simulink model "Buck_Parallel"  (R2023b)
settings: Solver=VariableStepAuto  StartTime=0.0  StopTime=0.03  RelTol=1e-3
libraries: spsSeriesRLCBranchLib x12, spsMosfetLib x11, spsCurrentMeasurementLib x9, simulink x6, spsVoltageMeasurementLib x6, slpidlib x6, spsDCVoltageSourceLib x2, spsControlledCurrentSourceLib x2, spsMeanLib x1, spsRMSLib x1, spspowerguiLib x1
settings Model: SimulationMode=accelerator  Creator=45276  LastModifiedBy=Epiphanye

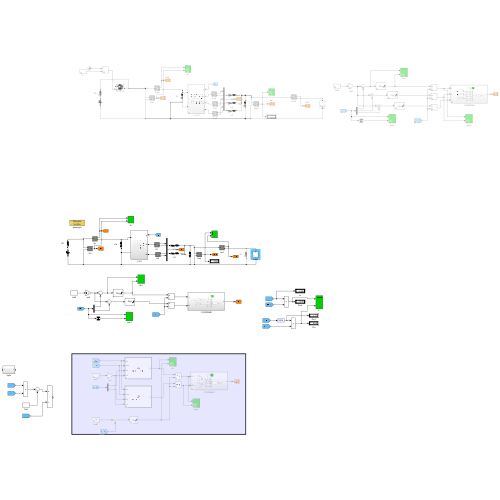
[thumbnail: Simulink's stored preview of the top-level diagram]
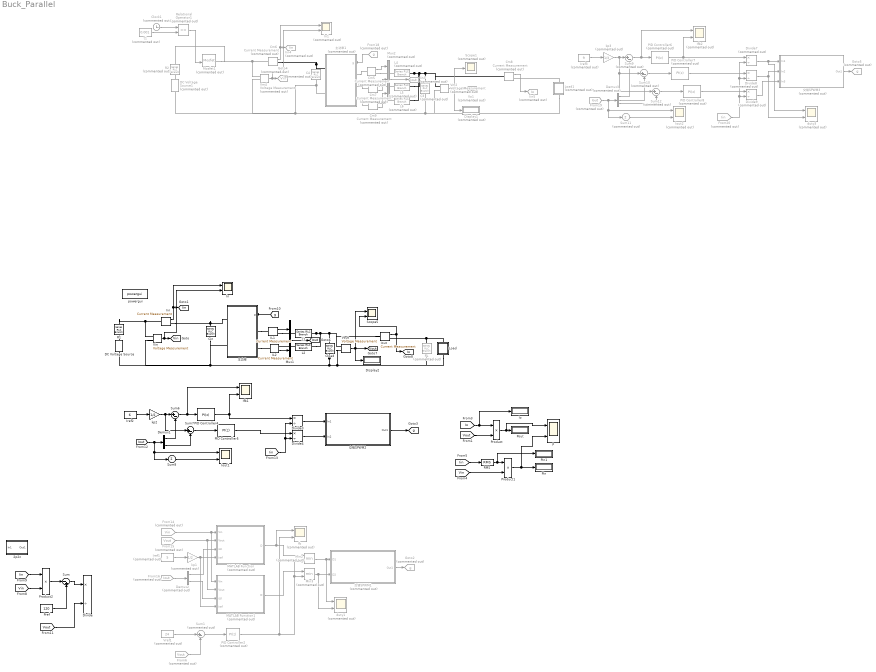
== system Buck_Parallel ==
  2p2z : Subsystem
  C3 : spsSeriesRLCBranchLib/Series RLC Branch  Commented=on  LConnTagsString=__new0  RConnTagsString=__new0  BranchType=RC  Resistance=0.015  Inductance=0  SetiL0=off  InitialCurrent=0  Capacitance=100e-6  Setx0=on  InitialVoltage=18  Measurements=None
  C4 : spsSeriesRLCBranchLib/Series RLC Branch  Commented=on  LConnTagsString=__new0  RConnTagsString=__new0  BranchType=RC  Resistance=0.01  Inductance=0  SetiL0=off  InitialCurrent=0  Capacitance=10e-6  Setx0=on  InitialVoltage=24  Measurements=None
  Cin : spsSeriesRLCBranchLib/Series RLC Branch  LConnTagsString=__new0  RConnTagsString=__new0  BranchType=RC  Resistance=0.15  Inductance=0  SetiL0=off  InitialCurrent=0  Capacitance=81e-6  Setx0=on  InitialVoltage=24  Measurements=None
  Cload : spsSeriesRLCBranchLib/Series RLC Branch  LConnTagsString=__new0  RConnTagsString=__new0  BranchType=RC  Resistance=0.018  Inductance=0  SetiL0=off  InitialCurrent=0  Capacitance=440e-6  Setx0=on  InitialVoltage=0  Measurements=None
  Clock1 : Clock  Commented=on
  Cm{5..9} (5 alike) : spsCurrentMeasurementLib/Current Measurement  Commented=on  PhasorSimulation=off  OutputType=Complex  PSBequivalent=0
  DC Voltage Source : spsDCVoltageSourceLib/DC Voltage Source  Amplitude=24  Measurements=None
  DC Voltage Source1 : spsDCVoltageSourceLib/DC Voltage Source  Commented=on  Amplitude=60  Measurements=None
  Demux1 : Demux  Outputs=2
  Demux2 : Demux  Commented=on  Outputs=2
  Demux3 : Demux  Commented=on  Outputs=3
  Display1 : Display  Commented=on
  Display2 : Display
  Divide : Product  Inputs=*/
  Divide3 : Product  Inputs=*/
  Divide4 : Product  Inputs=*/
  Divide7 : Product  Commented=on  Inputs=*/
  Divide8 : Product  Commented=on  Inputs=*/
  Divide9 : Product  Commented=on  Inputs=*/
  From14 : From  Commented=on  GotoTag=Vin  TagVisibility=global
      settings: CloseFcn=tagdialog Close
  From15 : From  Commented=on  GotoTag=Vout  TagVisibility=global
      settings: CloseFcn=tagdialog Close
  From16 : From  Commented=on  GotoTag=Iout  TagVisibility=global
      settings: CloseFcn=tagdialog Close
  From18 : From  Commented=on  GotoTag=g  TagVisibility=global
      settings: CloseFcn=tagdialog Close
  From19 : From  Commented=on  GotoTag=Iout  TagVisibility=global
      settings: CloseFcn=tagdialog Close
  From20 : From  Commented=on  GotoTag=Iin  TagVisibility=global
      settings: CloseFcn=tagdialog Close
  From6 : From  Commented=on  GotoTag=Vout  TagVisibility=global
      settings: CloseFcn=tagdialog Close
  Goto2 : Goto  Commented=on  GotoTag=g  TagVisibility=global
  Goto4 : Goto  Commented=on  GotoTag=Vin  TagVisibility=global
  Goto5 : Goto  Commented=on  GotoTag=g  TagVisibility=global
  IL1 : spsCurrentMeasurementLib/Current Measurement  PhasorSimulation=off  OutputType=Complex  PSBequivalent=0
  IL2 : spsCurrentMeasurementLib/Current Measurement  PhasorSimulation=off  OutputType=Complex  PSBequivalent=0
  Ifb1 : Scope  NumInputPorts=2
  Ifb2 : Scope  Commented=on  NumInputPorts=2
  Iin : spsCurrentMeasurementLib/Current Measurement  PhasorSimulation=off  OutputType=Complex  PSBequivalent=0
  Iin3 : Goto  Commented=on  GotoTag=Iout  TagVisibility=global
  Iin4 : Goto  Commented=on  GotoTag=Iin  TagVisibility=global
  Iin5 : Goto  Commented=on  GotoTag=Io  TagVisibility=global
  In : Scope  NumInputPorts=2
  In1 : Scope  Commented=on  NumInputPorts=2
  Io : Display
  Iout : spsCurrentMeasurementLib/Current Measurement  PhasorSimulation=off  OutputType=Complex  PSBequivalent=0
  Iout1 : Scope  NumInputPorts=2
  Iout2 : Scope  Commented=on  NumInputPorts=2
  Iref1 : Constant  Commented=on  Value=5
  Iref2 : Constant  Value=6
  Iref3 : Constant  Commented=on  Value=9
  L1 : spsSeriesRLCBranchLib/Series RLC Branch  LConnTagsString=__new0  RConnTagsString=__new0  BranchType=RL  Resistance=0.04  Inductance=221e-6  SetiL0=off  InitialCurrent=0  Capacitance=inf  Setx0=off  InitialVoltage=0  Measurements=None
  L2 : spsSeriesRLCBranchLib/Series RLC Branch  LConnTagsString=__new0  RConnTagsString=__new0  BranchType=RL  Resistance=0.04  Inductance=218e-6  SetiL0=off  InitialCurrent=0  Capacitance=inf  Setx0=off  InitialVoltage=0  Measurements=None
  L4 : spsSeriesRLCBranchLib/Series RLC Branch  Commented=on  LConnTagsString=__new0  RConnTagsString=__new0  BranchType=RL  Resistance=0.1  Inductance=4e-5  SetiL0=off  InitialCurrent=0  Capacitance=inf  Setx0=off  InitialVoltage=0  Measurements=None
  L5 : spsSeriesRLCBranchLib/Series RLC Branch  Commented=on  LConnTagsString=__new0  RConnTagsString=__new0  BranchType=RL  Resistance=0.1  Inductance=4e-5  SetiL0=off  InitialCurrent=0  Capacitance=inf  Setx0=off  InitialVoltage=0  Measurements=None
  L6 : spsSeriesRLCBranchLib/Series RLC Branch  Commented=on  LConnTagsString=__new0  RConnTagsString=__new0  BranchType=RL  Resistance=0.1  Inductance=4e-5  SetiL0=off  InitialCurrent=0  Capacitance=inf  Setx0=off  InitialVoltage=0  Measurements=None
  Load : Subsystem  mask{Vst1=[2 2 1 1 0.5 0.5].', Tst1=[0 0.01 0.01+eps 0.02 0.02+eps 0.03].', Tstsp=1e-8}
      mask prompts: Vst1 "突变值Vst1, eg:[3 3 8 8 2 2].'"; Tst1 "突变时间Tst1, eg:[0 0.01 0.01+eps 0.02 0.02+eps 0.03].'"; Tstsp "采样时间Tstsp"
      settings: PortSchema="{\"entries\":[{\"content\":{\"sides\":[{\"content\":{},\"type\":\"ConnectorPlacement.EquallySpacedRectSide\",\"uuid\":\"4352356a-a73d-4efd-aeba-c61bfc863045\"},{\"content\":{\"side\":\"RIGHT\"},\"type\":\"ConnectorPlacement.EquallySpacedRectSide\",\"uuid\":\"a043c14f-179e-462d-8cc8-5b83a7edcd21\"},{\"content\":{\"connectorIds\":[\"LConn1\"],\"side\":\"TOP\"},\"type\":\"ConnectorPlacement.EquallySpacedRectSide\",\"uuid\":\"f8810edc-586f-49c6-95ea-bd3a7aa2b56d\"},{\"content\":{\"connectorIds\":[\"RConn1\"],\"side\":\"BOTTOM\"},\"type\":\"ConnectorPlacement.EquallySpacedRectSide\",\"uuid\":\"956d2570-7b82-4c39-8513-d9bfab6f6be6\"}]},\"type\":\"ConnectorPlacement.EquallySpacedConnector\",\"uuid\":\"2f028cb1-1f36-487b-8c9b-3c22934b1877\"}],\"packageUris\":[\"http://schema.mathworks.com/mf0/Connector/R2020b\"],\"version\":\"1.0\"}"
      mask DialogControl ParameterGroupVar Prompt: 参数
  Load1 : Subsystem  Commented=on  mask{Vst1=[3 3 8 8 2 2].', Tst1=[0 0.01 0.01+eps 0.02 0.02+eps 0.03].', Tstsp=1e-8}
      mask prompts: Vst1 "突变值Vst1, eg:[3 3 8 8 2 2].'"; Tst1 "突变时间Tst1, eg:[0 0.01 0.01+eps 0.02 0.02+eps 0.03].'"; Tstsp "采样时间Tstsp"
      settings: PortSchema="{\"entries\":[{\"content\":{\"sides\":[{\"content\":{},\"type\":\"ConnectorPlacement.EquallySpacedRectSide\",\"uuid\":\"4352356a-a73d-4efd-aeba-c61bfc863045\"},{\"content\":{\"side\":\"RIGHT\"},\"type\":\"ConnectorPlacement.EquallySpacedRectSide\",\"uuid\":\"a043c14f-179e-462d-8cc8-5b83a7edcd21\"},{\"content\":{\"connectorIds\":[\"LConn1\"],\"side\":\"TOP\"},\"type\":\"ConnectorPlacement.EquallySpacedRectSide\",\"uuid\":\"f8810edc-586f-49c6-95ea-bd3a7aa2b56d\"},{\"content\":{\"connectorIds\":[\"RConn1\"],\"side\":\"BOTTOM\"},\"type\":\"ConnectorPlacement.EquallySpacedRectSide\",\"uuid\":\"956d2570-7b82-4c39-8513-d9bfab6f6be6\"}]},\"type\":\"ConnectorPlacement.EquallySpacedConnector\",\"uuid\":\"2f028cb1-1f36-487b-8c9b-3c22934b1877\"}],\"packageUris\":[\"http://schema.mathworks.com/mf0/Connector/R2020b\"],\"version\":\"1.0\"}"
      mask DialogControl ParameterGroupVar Prompt: 参数
  MATLAB Function : MATLAB Function  Commented=on  TreatAsAtomicUnit=on
  MATLAB Function1 : MATLAB Function  Commented=on  TreatAsAtomicUnit=on
  Min2 : MinMax  Commented=on  Inputs=2
  Min3 : MinMax  Commented=on  Inputs=2
  Mosfet1 : spsMosfetLib/Mosfet  Commented=on  Ron=0.1  Lon=0  Rd=0.01  Vfd=0  IC=0  Rs=1e5  Cs=inf  Measurements=off
  Mux1 : Mux  Inputs=2
  Mux2 : Mux  Commented=on  Inputs=3
  P : Scope  NumInputPorts=2
  PID Controller2 : slpidlib/PID Controller  Commented=on  Controller=PI  Form=Parallel  TimeDomain=Discrete-time  UseExternalTs=off  SampleTime=-1  IntegratorMethod=Forward Euler  FilterMethod=Forward Euler  ControllerParametersSource=internal  P=1.45  I=15  UseKiTs=off  D=0  N=100  UseFilter=on  TunerSelectOption=Transfer Function Based (PID Tuner App)  InitialConditionSource=internal  InitialConditionForIntegrator=0  InitialConditionForFilter=0  DifferentiatorICPrevScaledInput=0  ExternalReset=none  TrackingMode=off  Kt=100  LimitOutput=on  SatLimitsSource=internal  UpperSaturationLimit=1  LowerSaturationLimit=0  LinearizeAsGain=on  AntiWindupMode=clamping  Kb=1  LimitIntegrator=off  UpperIntegratorSaturationLimit=0.95  LowerIntegratorSaturationLimit=0  POutMin=[]  POutMax=[]  IOutMin=[]  IOutMax=[]  DOutMin=[]  DOutMax=[]  NOutMin=[]  NOutMax=[]  SumOutMin=[]  SumOutMax=[]  SaturationOutMin=[]  SaturationOutMax=[]  PParamMin=[]  PParamMax=[]  IParamMin=[]  IParamMax=[]  DParamMin=[]  DParamMax=[]  NParamMin=[]  NParamMax=[]  KbParamMin=[]  KbParamMax=[]  KtParamMin=[]  KtParamMax=[]  KbOutMin=[]  KbOutMax=[]  KtOutMin=[]  KtOutMax=[]  IntegratorOutMin=[]  IntegratorOutMax=[]  FilterOutMin=[]  FilterOutMax=[]  SumI1OutMin=[]  SumI1OutMax=[]  SumI2OutMin=[]  SumI2OutMax=[]  SumI3OutMin=[]  SumI3OutMax=[]  SumI4OutMin=[]  SumI4OutMax=[]  SumDOutMin=[]  SumDOutMax=[]  DifferentiatorOutMin=[]  DifferentiatorOutMax=[]  FilterDiffOutCoefMin=[]  FilterDiffOutCoefMax=[]  ReciprocalOutMin=[]  ReciprocalOutMax=[]  SumDenOutMin=[]  SumDenOutMax=[]  SumNumOutMin=[]  SumNumOutMax=[]  DivideOutMin=[]  DivideOutMax=[]  UdiffTsProdOutMin=[]  UdiffTsProdOutMax=[]  NTsProdOutMin=[]  NTsProdOutMax=[]  UintegralTsProdOutMin=[]  UintegralTsProdOutMax=[]  UngainTsProdOutMin=[]  UngainTsProdOutMax=[]  ClampingZeroOutDataTypeStr=Inherit: Inherit via back propagation  ClampingZeroOutMin=[]  ClampingZeroOutMax=[]  FilterDenConstantOutDataTypeStr=Inherit: Inherit via back propagation  FilterDenConstantOutMin=[]  FilterDenConstantOutMax=[]  PCopyOutDataTypeStr=Inherit: Inherit via back propagation  PCopyOutMin=[]  PCopyOutMax=[]  NCopyOutDataTypeStr=Inherit: Inherit via back propagation  NCopyOutMin=[]  NCopyOutMax=[]  IntegratorContinuousStateAttributes=''  IntegratorStateMustResolveToSignalObject=off  IntegratorRTWStateStorageClass=Auto  FilterContinuousStateAttributes=''  FilterStateMustResolveToSignalObject=off  FilterRTWStateStorageClass=Auto  ParallelPVariant=InternalParameters  IdealPVariant=Disabled  IVariant=InternalParameters  DVariant=Disabled  IntegratorVariant=Discrete  SatVariant=Enabled  AWVariant=DiscClampingParallel  PCopyVariant=Disabled  TRVariant=Disabled  FdbkBlocksVariant=Forward  IdealPFdbkVariant=Disabled  SatFdbkVariant=Disabled  DerivativeFilterVariant=Disabled  NVariant=Disabled  NCopyVariant=Disabled_SignalSpec  FilterICVariant=Disabled  IntegratorICVariant=InternalICs  ExternalResetVariant=Disabled  TRSumVariant=Passthrough  SumFdbkVariant=Disabled  SumVariant=Sum_PI  TsampFilterVariant=InternalTs  TsampNgainVariant=Passthrough  TsampIntegralVariant=Disabled_SignalSpec  ExternalSaturationOutDataTypeStr=Inherit: Same as second input
  PID Controller4 : slpidlib/PID Controller  Controller=PI  Form=Parallel  TimeDomain=Discrete-time  UseExternalTs=off  SampleTime=-1  IntegratorMethod=Forward Euler  FilterMethod=Forward Euler  ControllerParametersSource=internal  P=0.032  I=160  UseKiTs=off  D=0  N=100  UseFilter=on  TunerSelectOption=Transfer Function Based (PID Tuner App)  InitialConditionSource=internal  InitialConditionForIntegrator=0  InitialConditionForFilter=0  DifferentiatorICPrevScaledInput=0  ExternalReset=none  TrackingMode=off  Kt=1  LimitOutput=on  SatLimitsSource=internal  UpperSaturationLimit=1  LowerSaturationLimit=0  LinearizeAsGain=off  AntiWindupMode=clamping  Kb=1  LimitIntegrator=off  UpperIntegratorSaturationLimit=inf  LowerIntegratorSaturationLimit=-inf  POutMin=[]  POutMax=[]  IOutMin=[]  IOutMax=[]  DOutMin=[]  DOutMax=[]  NOutMin=[]  NOutMax=[]  SumOutMin=[]  SumOutMax=[]  SaturationOutMin=[]  SaturationOutMax=[]  PParamMin=[]  PParamMax=[]  IParamMin=[]  IParamMax=[]  DParamMin=[]  DParamMax=[]  NParamMin=[]  NParamMax=[]  KbParamMin=[]  KbParamMax=[]  KtParamMin=[]  KtParamMax=[]  KbOutMin=[]  KbOutMax=[]  KtOutMin=[]  KtOutMax=[]  IntegratorOutMin=[]  IntegratorOutMax=[]  FilterOutMin=[]  FilterOutMax=[]  SumI1OutMin=[]  SumI1OutMax=[]  SumI2OutMin=[]  SumI2OutMax=[]  SumI3OutMin=[]  SumI3OutMax=[]  SumI4OutMin=[]  SumI4OutMax=[]  SumDOutMin=[]  SumDOutMax=[]  DifferentiatorOutMin=[]  DifferentiatorOutMax=[]  FilterDiffOutCoefMin=[]  FilterDiffOutCoefMax=[]  ReciprocalOutMin=[]  ReciprocalOutMax=[]  SumDenOutMin=[]  SumDenOutMax=[]  SumNumOutMin=[]  SumNumOutMax=[]  DivideOutMin=[]  DivideOutMax=[]  UdiffTsProdOutMin=[]  UdiffTsProdOutMax=[]  NTsProdOutMin=[]  NTsProdOutMax=[]  UintegralTsProdOutMin=[]  UintegralTsProdOutMax=[]  UngainTsProdOutMin=[]  UngainTsProdOutMax=[]  ClampingZeroOutDataTypeStr=Inherit: Inherit via back propagation  ClampingZeroOutMin=[]  ClampingZeroOutMax=[]  FilterDenConstantOutDataTypeStr=Inherit: Inherit via back propagation  FilterDenConstantOutMin=[]  FilterDenConstantOutMax=[]  PCopyOutDataTypeStr=Inherit: Inherit via back propagation  PCopyOutMin=[]  PCopyOutMax=[]  NCopyOutDataTypeStr=Inherit: Inherit via back propagation  NCopyOutMin=[]  NCopyOutMax=[]  IntegratorContinuousStateAttributes=''  IntegratorStateMustResolveToSignalObject=off  IntegratorRTWStateStorageClass=Auto  FilterContinuousStateAttributes=''  FilterStateMustResolveToSignalObject=off  FilterRTWStateStorageClass=Auto  ParallelPVariant=InternalParameters  IdealPVariant=Disabled  IVariant=InternalParameters  DVariant=Disabled  IntegratorVariant=Discrete  SatVariant=Enabled  AWVariant=DiscClampingParallel  PCopyVariant=Disabled  TRVariant=Disabled  FdbkBlocksVariant=Forward  IdealPFdbkVariant=Disabled  SatFdbkVariant=Disabled  DerivativeFilterVariant=Disabled  NVariant=Disabled  NCopyVariant=Disabled_SignalSpec  FilterICVariant=Disabled  IntegratorICVariant=InternalICs  ExternalResetVariant=Disabled  TRSumVariant=Passthrough  SumFdbkVariant=Disabled  SumVariant=Sum_PI  TsampFilterVariant=InternalTs  TsampNgainVariant=Passthrough  TsampIntegralVariant=Disabled_SignalSpec  ExternalSaturationOutDataTypeStr=Inherit: Same as second input
  PID Controller5 : slpidlib/PID Controller  Controller=PI  Form=Parallel  TimeDomain=Discrete-time  UseExternalTs=off  SampleTime=-1  IntegratorMethod=Forward Euler  FilterMethod=Forward Euler  ControllerParametersSource=internal  P=0.032  I=160  UseKiTs=off  D=0  N=100  UseFilter=on  TunerSelectOption=Transfer Function Based (PID Tuner App)  InitialConditionSource=internal  InitialConditionForIntegrator=0  InitialConditionForFilter=0  DifferentiatorICPrevScaledInput=0  ExternalReset=none  TrackingMode=off  Kt=1  LimitOutput=on  SatLimitsSource=internal  UpperSaturationLimit=1  LowerSaturationLimit=0  LinearizeAsGain=off  AntiWindupMode=clamping  Kb=1  LimitIntegrator=off  UpperIntegratorSaturationLimit=inf  LowerIntegratorSaturationLimit=-inf  POutMin=[]  POutMax=[]  IOutMin=[]  IOutMax=[]  DOutMin=[]  DOutMax=[]  NOutMin=[]  NOutMax=[]  SumOutMin=[]  SumOutMax=[]  SaturationOutMin=[]  SaturationOutMax=[]  PParamMin=[]  PParamMax=[]  IParamMin=[]  IParamMax=[]  DParamMin=[]  DParamMax=[]  NParamMin=[]  NParamMax=[]  KbParamMin=[]  KbParamMax=[]  KtParamMin=[]  KtParamMax=[]  KbOutMin=[]  KbOutMax=[]  KtOutMin=[]  KtOutMax=[]  IntegratorOutMin=[]  IntegratorOutMax=[]  FilterOutMin=[]  FilterOutMax=[]  SumI1OutMin=[]  SumI1OutMax=[]  SumI2OutMin=[]  SumI2OutMax=[]  SumI3OutMin=[]  SumI3OutMax=[]  SumI4OutMin=[]  SumI4OutMax=[]  SumDOutMin=[]  SumDOutMax=[]  DifferentiatorOutMin=[]  DifferentiatorOutMax=[]  FilterDiffOutCoefMin=[]  FilterDiffOutCoefMax=[]  ReciprocalOutMin=[]  ReciprocalOutMax=[]  SumDenOutMin=[]  SumDenOutMax=[]  SumNumOutMin=[]  SumNumOutMax=[]  DivideOutMin=[]  DivideOutMax=[]  UdiffTsProdOutMin=[]  UdiffTsProdOutMax=[]  NTsProdOutMin=[]  NTsProdOutMax=[]  UintegralTsProdOutMin=[]  UintegralTsProdOutMax=[]  UngainTsProdOutMin=[]  UngainTsProdOutMax=[]  ClampingZeroOutDataTypeStr=Inherit: Inherit via back propagation  ClampingZeroOutMin=[]  ClampingZeroOutMax=[]  FilterDenConstantOutDataTypeStr=Inherit: Inherit via back propagation  FilterDenConstantOutMin=[]  FilterDenConstantOutMax=[]  PCopyOutDataTypeStr=Inherit: Inherit via back propagation  PCopyOutMin=[]  PCopyOutMax=[]  NCopyOutDataTypeStr=Inherit: Inherit via back propagation  NCopyOutMin=[]  NCopyOutMax=[]  IntegratorContinuousStateAttributes=''  IntegratorStateMustResolveToSignalObject=off  IntegratorRTWStateStorageClass=Auto  FilterContinuousStateAttributes=''  FilterStateMustResolveToSignalObject=off  FilterRTWStateStorageClass=Auto  ParallelPVariant=InternalParameters  IdealPVariant=Disabled  IVariant=InternalParameters  DVariant=Disabled  IntegratorVariant=Discrete  SatVariant=Enabled  AWVariant=DiscClampingParallel  PCopyVariant=Disabled  TRVariant=Disabled  FdbkBlocksVariant=Forward  IdealPFdbkVariant=Disabled  SatFdbkVariant=Disabled  DerivativeFilterVariant=Disabled  NVariant=Disabled  NCopyVariant=Disabled_SignalSpec  FilterICVariant=Disabled  IntegratorICVariant=InternalICs  ExternalResetVariant=Disabled  TRSumVariant=Passthrough  SumFdbkVariant=Disabled  SumVariant=Sum_PI  TsampFilterVariant=InternalTs  TsampNgainVariant=Passthrough  TsampIntegralVariant=Disabled_SignalSpec  ExternalSaturationOutDataTypeStr=Inherit: Same as second input
  PID Controller6 : slpidlib/PID Controller  Commented=on  Controller=PI  Form=Parallel  TimeDomain=Discrete-time  UseExternalTs=off  SampleTime=-1  IntegratorMethod=Forward Euler  FilterMethod=Forward Euler  ControllerParametersSource=internal  P=1  I=1  UseKiTs=off  D=0  N=100  UseFilter=on  TunerSelectOption=Transfer Function Based (PID Tuner App)  InitialConditionSource=internal  InitialConditionForIntegrator=0  InitialConditionForFilter=0  DifferentiatorICPrevScaledInput=0  ExternalReset=none  TrackingMode=off  Kt=1  LimitOutput=on  SatLimitsSource=internal  UpperSaturationLimit=1  LowerSaturationLimit=0  LinearizeAsGain=off  AntiWindupMode=clamping  Kb=1  LimitIntegrator=off  UpperIntegratorSaturationLimit=inf  LowerIntegratorSaturationLimit=-inf  POutMin=[]  POutMax=[]  IOutMin=[]  IOutMax=[]  DOutMin=[]  DOutMax=[]  NOutMin=[]  NOutMax=[]  SumOutMin=[]  SumOutMax=[]  SaturationOutMin=[]  SaturationOutMax=[]  PParamMin=[]  PParamMax=[]  IParamMin=[]  IParamMax=[]  DParamMin=[]  DParamMax=[]  NParamMin=[]  NParamMax=[]  KbParamMin=[]  KbParamMax=[]  KtParamMin=[]  KtParamMax=[]  KbOutMin=[]  KbOutMax=[]  KtOutMin=[]  KtOutMax=[]  IntegratorOutMin=[]  IntegratorOutMax=[]  FilterOutMin=[]  FilterOutMax=[]  SumI1OutMin=[]  SumI1OutMax=[]  SumI2OutMin=[]  SumI2OutMax=[]  SumI3OutMin=[]  SumI3OutMax=[]  SumI4OutMin=[]  SumI4OutMax=[]  SumDOutMin=[]  SumDOutMax=[]  DifferentiatorOutMin=[]  DifferentiatorOutMax=[]  FilterDiffOutCoefMin=[]  FilterDiffOutCoefMax=[]  ReciprocalOutMin=[]  ReciprocalOutMax=[]  SumDenOutMin=[]  SumDenOutMax=[]  SumNumOutMin=[]  SumNumOutMax=[]  DivideOutMin=[]  DivideOutMax=[]  UdiffTsProdOutMin=[]  UdiffTsProdOutMax=[]  NTsProdOutMin=[]  NTsProdOutMax=[]  UintegralTsProdOutMin=[]  UintegralTsProdOutMax=[]  UngainTsProdOutMin=[]  UngainTsProdOutMax=[]  ClampingZeroOutDataTypeStr=Inherit: Inherit via back propagation  ClampingZeroOutMin=[]  ClampingZeroOutMax=[]  FilterDenConstantOutDataTypeStr=Inherit: Inherit via back propagation  FilterDenConstantOutMin=[]  FilterDenConstantOutMax=[]  PCopyOutDataTypeStr=Inherit: Inherit via back propagation  PCopyOutMin=[]  PCopyOutMax=[]  NCopyOutDataTypeStr=Inherit: Inherit via back propagation  NCopyOutMin=[]  NCopyOutMax=[]  IntegratorContinuousStateAttributes=''  IntegratorStateMustResolveToSignalObject=off  IntegratorRTWStateStorageClass=Auto  FilterContinuousStateAttributes=''  FilterStateMustResolveToSignalObject=off  FilterRTWStateStorageClass=Auto  ParallelPVariant=InternalParameters  IdealPVariant=Disabled  IVariant=InternalParameters  DVariant=Disabled  IntegratorVariant=Discrete  SatVariant=Enabled  AWVariant=DiscClampingParallel  PCopyVariant=Disabled  TRVariant=Disabled  FdbkBlocksVariant=Forward  IdealPFdbkVariant=Disabled  SatFdbkVariant=Disabled  DerivativeFilterVariant=Disabled  NVariant=Disabled  NCopyVariant=Disabled_SignalSpec  FilterICVariant=Disabled  IntegratorICVariant=InternalICs  ExternalResetVariant=Disabled  TRSumVariant=Passthrough  SumFdbkVariant=Disabled  SumVariant=Sum_PI  TsampFilterVariant=InternalTs  TsampNgainVariant=Passthrough  TsampIntegralVariant=Disabled_SignalSpec  ExternalSaturationOutDataTypeStr=Inherit: Same as second input
  PID Controller7 : slpidlib/PID Controller  Commented=on  Controller=PI  Form=Parallel  TimeDomain=Discrete-time  UseExternalTs=off  SampleTime=-1  IntegratorMethod=Forward Euler  FilterMethod=Forward Euler  ControllerParametersSource=internal  P=1  I=1  UseKiTs=off  D=0  N=100  UseFilter=on  TunerSelectOption=Transfer Function Based (PID Tuner App)  InitialConditionSource=internal  InitialConditionForIntegrator=0  InitialConditionForFilter=0  DifferentiatorICPrevScaledInput=0  ExternalReset=none  TrackingMode=off  Kt=1  LimitOutput=on  SatLimitsSource=internal  UpperSaturationLimit=1  LowerSaturationLimit=0  LinearizeAsGain=off  AntiWindupMode=clamping  Kb=1  LimitIntegrator=off  UpperIntegratorSaturationLimit=inf  LowerIntegratorSaturationLimit=-inf  POutMin=[]  POutMax=[]  IOutMin=[]  IOutMax=[]  DOutMin=[]  DOutMax=[]  NOutMin=[]  NOutMax=[]  SumOutMin=[]  SumOutMax=[]  SaturationOutMin=[]  SaturationOutMax=[]  PParamMin=[]  PParamMax=[]  IParamMin=[]  IParamMax=[]  DParamMin=[]  DParamMax=[]  NParamMin=[]  NParamMax=[]  KbParamMin=[]  KbParamMax=[]  KtParamMin=[]  KtParamMax=[]  KbOutMin=[]  KbOutMax=[]  KtOutMin=[]  KtOutMax=[]  IntegratorOutMin=[]  IntegratorOutMax=[]  FilterOutMin=[]  FilterOutMax=[]  SumI1OutMin=[]  SumI1OutMax=[]  SumI2OutMin=[]  SumI2OutMax=[]  SumI3OutMin=[]  SumI3OutMax=[]  SumI4OutMin=[]  SumI4OutMax=[]  SumDOutMin=[]  SumDOutMax=[]  DifferentiatorOutMin=[]  DifferentiatorOutMax=[]  FilterDiffOutCoefMin=[]  FilterDiffOutCoefMax=[]  ReciprocalOutMin=[]  ReciprocalOutMax=[]  SumDenOutMin=[]  SumDenOutMax=[]  SumNumOutMin=[]  SumNumOutMax=[]  DivideOutMin=[]  DivideOutMax=[]  UdiffTsProdOutMin=[]  UdiffTsProdOutMax=[]  NTsProdOutMin=[]  NTsProdOutMax=[]  UintegralTsProdOutMin=[]  UintegralTsProdOutMax=[]  UngainTsProdOutMin=[]  UngainTsProdOutMax=[]  ClampingZeroOutDataTypeStr=Inherit: Inherit via back propagation  ClampingZeroOutMin=[]  ClampingZeroOutMax=[]  FilterDenConstantOutDataTypeStr=Inherit: Inherit via back propagation  FilterDenConstantOutMin=[]  FilterDenConstantOutMax=[]  PCopyOutDataTypeStr=Inherit: Inherit via back propagation  PCopyOutMin=[]  PCopyOutMax=[]  NCopyOutDataTypeStr=Inherit: Inherit via back propagation  NCopyOutMin=[]  NCopyOutMax=[]  IntegratorContinuousStateAttributes=''  IntegratorStateMustResolveToSignalObject=off  IntegratorRTWStateStorageClass=Auto  FilterContinuousStateAttributes=''  FilterStateMustResolveToSignalObject=off  FilterRTWStateStorageClass=Auto  ParallelPVariant=InternalParameters  IdealPVariant=Disabled  IVariant=InternalParameters  DVariant=Disabled  IntegratorVariant=Discrete  SatVariant=Enabled  AWVariant=DiscClampingParallel  PCopyVariant=Disabled  TRVariant=Disabled  FdbkBlocksVariant=Forward  IdealPFdbkVariant=Disabled  SatFdbkVariant=Disabled  DerivativeFilterVariant=Disabled  NVariant=Disabled  NCopyVariant=Disabled_SignalSpec  FilterICVariant=Disabled  IntegratorICVariant=InternalICs  ExternalResetVariant=Disabled  TRSumVariant=Passthrough  SumFdbkVariant=Disabled  SumVariant=Sum_PI  TsampFilterVariant=InternalTs  TsampNgainVariant=Passthrough  TsampIntegralVariant=Disabled_SignalSpec  ExternalSaturationOutDataTypeStr=Inherit: Same as second input
  PID Controller8 : slpidlib/PID Controller  Commented=on  Controller=PI  Form=Parallel  TimeDomain=Discrete-time  UseExternalTs=off  SampleTime=-1  IntegratorMethod=Forward Euler  FilterMethod=Forward Euler  ControllerParametersSource=internal  P=1  I=1  UseKiTs=off  D=0  N=100  UseFilter=on  TunerSelectOption=Transfer Function Based (PID Tuner App)  InitialConditionSource=internal  InitialConditionForIntegrator=0  InitialConditionForFilter=0  DifferentiatorICPrevScaledInput=0  ExternalReset=none  TrackingMode=off  Kt=1  LimitOutput=on  SatLimitsSource=internal  UpperSaturationLimit=1  LowerSaturationLimit=0  LinearizeAsGain=off  AntiWindupMode=clamping  Kb=1  LimitIntegrator=off  UpperIntegratorSaturationLimit=inf  LowerIntegratorSaturationLimit=-inf  POutMin=[]  POutMax=[]  IOutMin=[]  IOutMax=[]  DOutMin=[]  DOutMax=[]  NOutMin=[]  NOutMax=[]  SumOutMin=[]  SumOutMax=[]  SaturationOutMin=[]  SaturationOutMax=[]  PParamMin=[]  PParamMax=[]  IParamMin=[]  IParamMax=[]  DParamMin=[]  DParamMax=[]  NParamMin=[]  NParamMax=[]  KbParamMin=[]  KbParamMax=[]  KtParamMin=[]  KtParamMax=[]  KbOutMin=[]  KbOutMax=[]  KtOutMin=[]  KtOutMax=[]  IntegratorOutMin=[]  IntegratorOutMax=[]  FilterOutMin=[]  FilterOutMax=[]  SumI1OutMin=[]  SumI1OutMax=[]  SumI2OutMin=[]  SumI2OutMax=[]  SumI3OutMin=[]  SumI3OutMax=[]  SumI4OutMin=[]  SumI4OutMax=[]  SumDOutMin=[]  SumDOutMax=[]  DifferentiatorOutMin=[]  DifferentiatorOutMax=[]  FilterDiffOutCoefMin=[]  FilterDiffOutCoefMax=[]  ReciprocalOutMin=[]  ReciprocalOutMax=[]  SumDenOutMin=[]  SumDenOutMax=[]  SumNumOutMin=[]  SumNumOutMax=[]  DivideOutMin=[]  DivideOutMax=[]  UdiffTsProdOutMin=[]  UdiffTsProdOutMax=[]  NTsProdOutMin=[]  NTsProdOutMax=[]  UintegralTsProdOutMin=[]  UintegralTsProdOutMax=[]  UngainTsProdOutMin=[]  UngainTsProdOutMax=[]  ClampingZeroOutDataTypeStr=Inherit: Inherit via back propagation  ClampingZeroOutMin=[]  ClampingZeroOutMax=[]  FilterDenConstantOutDataTypeStr=Inherit: Inherit via back propagation  FilterDenConstantOutMin=[]  FilterDenConstantOutMax=[]  PCopyOutDataTypeStr=Inherit: Inherit via back propagation  PCopyOutMin=[]  PCopyOutMax=[]  NCopyOutDataTypeStr=Inherit: Inherit via back propagation  NCopyOutMin=[]  NCopyOutMax=[]  IntegratorContinuousStateAttributes=''  IntegratorStateMustResolveToSignalObject=off  IntegratorRTWStateStorageClass=Auto  FilterContinuousStateAttributes=''  FilterStateMustResolveToSignalObject=off  FilterRTWStateStorageClass=Auto  ParallelPVariant=InternalParameters  IdealPVariant=Disabled  IVariant=InternalParameters  DVariant=Disabled  IntegratorVariant=Discrete  SatVariant=Enabled  AWVariant=DiscClampingParallel  PCopyVariant=Disabled  TRVariant=Disabled  FdbkBlocksVariant=Forward  IdealPFdbkVariant=Disabled  SatFdbkVariant=Disabled  DerivativeFilterVariant=Disabled  NVariant=Disabled  NCopyVariant=Disabled_SignalSpec  FilterICVariant=Disabled  IntegratorICVariant=InternalICs  ExternalResetVariant=Disabled  TRSumVariant=Passthrough  SumFdbkVariant=Disabled  SumVariant=Sum_PI  TsampFilterVariant=InternalTs  TsampNgainVariant=Passthrough  TsampIntegralVariant=Disabled_SignalSpec  ExternalSaturationOutDataTypeStr=Inherit: Same as second input
  Pin : Display
  Pin1 : Display
  Pout : Display
  Pref : Constant  Value=120
  Product : Product
  Product1 : Product
  Product2 : Product
  R1 : spsSeriesRLCBranchLib/Series RLC Branch  LConnTagsString=__new0  RConnTagsString=__new0  BranchType=R  Resistance=0.01  Inductance=0  SetiL0=off  InitialCurrent=0  Capacitance=10e-6  Setx0=on  InitialVoltage=24  Measurements=None
  R2 : spsSeriesRLCBranchLib/Series RLC Branch  Commented=on  LConnTagsString=__new0  RConnTagsString=__new0  BranchType=R  Resistance=0.01  Inductance=0  SetiL0=off  InitialCurrent=0  Capacitance=10e-6  Setx0=on  InitialVoltage=24  Measurements=None
  RL : spsSeriesRLCBranchLib/Series RLC Branch  Commented=on  LConnTagsString=__new0  RConnTagsString=__new0  BranchType=R  Resistance=0.5  Inductance=0  SetiL0=off  InitialCurrent=0  Capacitance=440e-6  Setx0=on  InitialVoltage=10  Measurements=None
  RMS : spsRMSLib/RMS  TrueRMS=on  Freq=60  RMSInit=120  Ts=0
  Relational Operator1 : RelationalOperator  Commented=on  OutDataTypeStr=boolean  InputSameDT=off
  Scope1 : Scope  Commented=on
  Scope5 : Scope  NumInputPorts=2
  Sum : Sum  Inputs=|-+
  Sum{1,9..10,12} (4 alike) : Sum  Commented=on  Inputs=|+-
  Sum11 : Sum  Commented=on  Inputs=+
  Sum6 : Sum  Inputs=|+-
  Sum7 : Sum  Inputs=|+-
  Sum8 : Sum  Inputs=+
  Vin : spsVoltageMeasurementLib/Voltage Measurement  PhasorSimulation=off  OutputType=Complex  PSBequivalent=0
  Vm2 : spsVoltageMeasurementLib/Voltage Measurement  Commented=on  PhasorSimulation=off  OutputType=Complex  PSBequivalent=0
  Vm4 : spsVoltageMeasurementLib/Voltage Measurement  Commented=on  PhasorSimulation=off  OutputType=Complex  PSBequivalent=0
  Vo1 : Goto  Commented=on  GotoTag=Vout  TagVisibility=global
  Vout : spsVoltageMeasurementLib/Voltage Measurement  PhasorSimulation=off  OutputType=Complex  PSBequivalent=0
  Vref1 : Constant  Commented=on  Value=24
  duty1 : Scope  Commented=on  NumInputPorts=2
  duty3 : Scope  Commented=on  NumInputPorts=2
  fb : Scope  Commented=on  NumInputPorts=2
  kp1 : Gain  Commented=on  Gain=1/2
  kp2 : Gain  Gain=1/2
  kp3 : Gain  Commented=on  Gain=1/3
  powergui : spspowerguiLib/powergui  SimulationMode=Discrete  SampleTime=1e-8  frequency=60  Iterations=50  frequencyindice=0  Pbase=100e6  ErrMax=1e-4  UnitsV=kV  UnitsW=MW  buscounter=0  FunctionMessages=off  echomessages=off  EnableUseOfTLC=off  CurrentSourceSwitches=off  DisableSnubberDevices=off  DisableRonSwitches=off  DisableVfSwitches=off  DisplayEquations=off  AutomaticDiscreteSolvers=off  SolverType=Tustin/Backward Euler (TBE)  Interpol=off  ExternalGateDelay=off  methode=off  Ts=0  x0status=blocks  SPID=off  SwTol=0  HookPort=off  NonlinearTolerance=1e-4  nMaxIteration=100  ContinueOnMaxIteration=off  RestoreLinks=warning  ResistiveCurrentMeasurement=off  Frange=[0:2:500]  Ylog=off  Xlog=on  ShowGrid=off  save=off  variable=ZData  structure=QQQQQ  ZoomFFT=off  StartTime=0.5  cycles=15  DisplayStyle=1  fundamental=50  FreqAxis=off  MaxFrequency=1000  frequencyindicesteady=1  RmsSteady=1  display=off
  t1 : Constant  Commented=on  Value=0.001
  主功率 : Subsystem
      settings: PortSchema="{\"entries\":[{\"content\":{\"sides\":[{\"content\":{\"connectorIds\":[\"LConn1\",\"LConn2\"]},\"type\":\"ConnectorPlacement.EquallySpacedRectSide\",\"uuid\":\"ac97cf15-7e99-4aeb-9e40-9a28a417beb8\"},{\"content\":{\"connectorIds\":[\"In1\",\"RConn1\",\"RConn2\"],\"side\":\"RIGHT\"},\"type\":\"ConnectorPlacement.EquallySpacedRectSide\",\"uuid\":\"b75e0bc0-5f77-40b8-af09-cbcb0210c65c\"},{\"content\":{\"side\":\"TOP\"},\"type\":\"ConnectorPlacement.EquallySpacedRectSide\",\"uuid\":\"53bad155-123f-4f3b-80a9-0e1646e28bdc\"}]},\"type\":\"ConnectorPlacement.EquallySpacedConnector\",\"uuid\":\"bded8531-36b4-4dbd-93e6-ef6e40a74a78\"}],\"packageUris\":[\"http://schema.mathworks.com/mf0/Connector/R2020b\"],\"version\":\"1.0\"}"
  主功率1 : Subsystem  Commented=on
      settings: PortSchema="{\"entries\":[{\"content\":{\"sides\":[{\"content\":{\"connectorIds\":[\"LConn1\",\"LConn2\"]},\"type\":\"ConnectorPlacement.EquallySpacedRectSide\",\"uuid\":\"ac97cf15-7e99-4aeb-9e40-9a28a417beb8\"},{\"content\":{\"connectorIds\":[\"In1\",\"RConn1\",\"RConn2\",\"RConn3\"],\"side\":\"RIGHT\"},\"type\":\"ConnectorPlacement.EquallySpacedRectSide\",\"uuid\":\"b75e0bc0-5f77-40b8-af09-cbcb0210c65c\"},{\"content\":{\"side\":\"TOP\"},\"type\":\"ConnectorPlacement.EquallySpacedRectSide\",\"uuid\":\"53bad155-123f-4f3b-80a9-0e1646e28bdc\"}]},\"type\":\"ConnectorPlacement.EquallySpacedConnector\",\"uuid\":\"bded8531-36b4-4dbd-93e6-ef6e40a74a78\"}],\"packageUris\":[\"http://schema.mathworks.com/mf0/Connector/R2020b\"],\"version\":\"1.0\"}"
  交错SPWM1 : Subsystem  Commented=on
  交错SPWM2 : Subsystem
  交错SPWM3 : Subsystem  Commented=on
  tag scope: Iin=global, Io=global, Iout=global, Vin=global, Vout=global, g=global
  wires:
  Product/1 -> P/1, Pout/1
  Mux1/1 -> [Iout]
  [Io] -> Io/1, Product/1
  [Vout] -> Product/2
  [g] -> 主功率/1(g)
  IL1/1 -> Mux1/1
  Vout/1 -> Display2/1, Scope5/1, [Vout]
  Vin/1 -> In/2, [Vin]
  IL2/1 -> Mux1/2
  Iin/1 -> In/1, [Iin]
  [Vin] -> Product1/2
  Iout/1 -> Scope5/2, [Io]
  Product1/1 -> P/2, Pin/1
  [Iin] -> Product2/1
  [Vin] -> Product2/2
  Product2/1 -> Sum/1
  Pref/1 -> Sum/2
  Sum/1 -> Divide/1
  [Vout] -> Divide/2
  From14/1 -> MATLAB Function1/1(Vin), MATLAB Function/1(Vin)
  From15/1 -> MATLAB Function1/2(Vout), MATLAB Function/2(Vout)
  From16/1 -> Demux2/1
  Demux2/1 -> MATLAB Function/3(iLK)
  Iref1/1 -> kp1/1
  kp1/1 -> MATLAB Function1/4(Iref), MATLAB Function/4(Iref)
  Demux2/2 -> MATLAB Function1/3(iLK)
  交错SPWM1/1(Out1) -> Goto2/1
  Min2/1 -> duty1/1, 交错SPWM1/1(D1)
  Min3/1 -> duty1/2, 交错SPWM1/2(D2)
  MATLAB Function/1(D) -> fb/1, Min2/1
  MATLAB Function1/1(D) -> Min3/1
  Vref1/1 -> Sum1/1
  Sum1/1 -> PID Controller2/1
  From6/1 -> Sum1/2
  PID Controller2/1 -> fb/2, Min3/2, Min2/2
  [Iin] -> Divide3/2, Divide4/2
  PID Controller5/1 -> Divide4/1
  PID Controller4/1 -> Divide3/1, Ifb1/2
  Iref2/1 -> kp2/1
  [Iout] -> Demux1/1, Iout1/1, Sum8/1
  Sum6/1 -> PID Controller4/1, Ifb1/1
  交错SPWM2/1(Out1) -> [g]
  Sum8/1 -> Iout1/2
  Sum7/1 -> PID Controller5/1
  Demux1/1 -> Sum6/2
  Demux1/2 -> Sum7/2
  kp2/1 -> Sum6/1, Sum7/1
  Relational Operator1/1 -> Mosfet1/1
  t1/1 -> Relational Operator1/2
  Clock1/1 -> Relational Operator1/1
  Cm8/1 -> Iin5/1
  Cm6/1 -> Iin4/1, In1/1
  Cm7/1 -> Mux2/2
  Vm4/1 -> Goto4/1, In1/2
  Vm2/1 -> Vo1/1, Scope1/1, Display1/1
  Cm5/1 -> Mux2/1
  From18/1 -> 主功率1/1(g)
  Mux2/1 -> Iin3/1
  Cm9/1 -> Mux2/3
  kp3/1 -> Sum12/1, Sum10/1, Sum9/1
  Demux3/2 -> Sum10/2
  Demux3/1 -> Sum9/2
  Sum10/1 -> PID Controller7/1
  Sum11/1 -> Iout2/2
  交错SPWM3/1(Out1) -> Goto5/1
  Sum9/1 -> Ifb2/1, PID Controller6/1
  From19/1 -> Sum11/1, Iout2/1, Demux3/1
  Iref3/1 -> kp3/1
  PID Controller6/1 -> Ifb2/2, Divide7/1
  Divide7/1 -> duty3/1, 交错SPWM3/1(In1)
  PID Controller7/1 -> Divide8/1
  Divide8/1 -> duty3/2, 交错SPWM3/2(In2)
  From20/1 -> Divide9/2, Divide8/2, Divide7/2
  Divide9/1 -> 交错SPWM3/3(In3)
  Sum12/1 -> PID Controller8/1
  Demux3/3 -> Sum12/2
  PID Controller8/1 -> Divide9/1
  [Iin] -> RMS/1
  RMS/1 -> Pin1/1, Product1/1
  Divide3/1 -> 交错SPWM2/1(In1)
  Divide4/1 -> 交错SPWM2/2(In2)
  connections:
  L1/RConn1 -- Iout/LConn1 -- Vout/LConn1 -- Cload/LConn1 -- L2/RConn1
  Iin/LConn1 -- R1/LConn1 -- Vin/LConn1
  主功率/RConn2 -- IL2/LConn1
  L2/LConn1 -- IL2/RConn1
  IL1/RConn1 -- L1/LConn1
  主功率/RConn1 -- IL1/LConn1
  DC Voltage Source/RConn1 -- R1/RConn1
  Cload/RConn1 -- Vin/LConn2 -- DC Voltage Source/LConn1 -- Cin/RConn1 -- 主功率/LConn2 -- RL/RConn1 -- Load/RConn1 -- Vout/LConn2
  Load/LConn1 -- RL/LConn1 -- Iout/RConn1
  L4/RConn1 -- L6/RConn1 -- L5/RConn1 -- C3/LConn1 -- Vm2/LConn1 -- Cm8/LConn1
  Cm6/LConn1 -- Vm4/LConn1 -- Mosfet1/RConn1 -- R2/LConn1
  C4/RConn1 -- 主功率1/LConn2 -- DC Voltage Source1/LConn1 -- Vm4/LConn2 -- Load1/RConn1 -- Vm2/LConn2 -- C3/RConn1
  C4/LConn1 -- Cm6/RConn1 -- 主功率1/LConn1
  Load1/LConn1 -- Cm8/RConn1
  DC Voltage Source1/RConn1 -- R2/RConn1
  主功率1/RConn2 -- Cm7/LConn1
  L5/LConn1 -- Cm7/RConn1
  Cm5/RConn1 -- L4/LConn1
  主功率1/RConn1 -- Cm5/LConn1
  Cm9/LConn1 -- 主功率1/RConn3
  Cm9/RConn1 -- L6/LConn1
  Iin/RConn1 -- Cin/LConn1 -- 主功率/LConn1

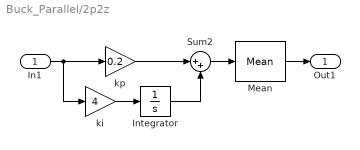
== system Buck_Parallel/2p2z ==
  In1 : Inport
  Integrator : Integrator  LimitOutput=on  UpperSaturationLimit=0.98  LowerSaturationLimit=0
  Mean : spsMeanLib/Mean  Freq=10000  Vinit=0  Ts=0
  Sum2 : Sum  Inputs=|++
  ki : Gain  Gain=4
  kp : Gain  Gain=0.2
  Out1 : Outport
  wires:
  In1/1 -> ki/1, kp/1
  ki/1 -> Integrator/1
  kp/1 -> Sum2/1
  Integrator/1 -> Sum2/2
  Sum2/1 -> Mean/1
  Mean/1 -> Out1/1

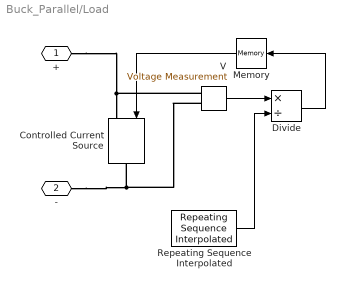
== system Buck_Parallel/Load ==
  Controlled Current Source : spsControlledCurrentSourceLib/Controlled Current Source  Initialize=on  Source_Type=AC  Amplitude=0  Phase=0  Frequency=0  Measurements=None
  Divide : Product  Inputs=*/
  Memory : Memory
  Repeating Sequence Interpolated : simulink/Sources/Repeating Sequence Interpolated  OutValues=Vst1  TimeValues=Tst1  LookUpMeth=Interpolation-Use End Values  tsamp=Tstsp  OutMin=[]  OutMax=[]  OutDataTypeStr=double  OutputDataTypeScalingMode=double  OutDataType=fixdt(0,8)  OutScaling=2^-10
  V : spsVoltageMeasurementLib/Voltage Measurement  PhasorSimulation=off  OutputType=Complex  PSBequivalent=0
  + : PMIOPort  Side=Left
  - : PMIOPort  Port=2  Side=Right
  wires:
  V/1 -> Divide/1
  Divide/1 -> Memory/1
  Repeating Sequence Interpolated/1 -> Divide/2
  Memory/1 -> Controlled Current Source/1
  connections:
  V/LConn1 -- Controlled Current Source/LConn1 -- +/RConn1
  V/LConn2 -- -/RConn1 -- Controlled Current Source/RConn1

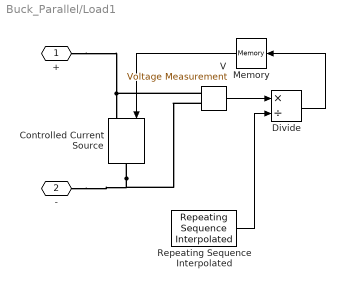
== system Buck_Parallel/Load1 ==
  Controlled Current Source : spsControlledCurrentSourceLib/Controlled Current Source  Initialize=on  Source_Type=AC  Amplitude=0  Phase=0  Frequency=0  Measurements=None
  Divide : Product  Inputs=*/
  Memory : Memory
  Repeating Sequence Interpolated : simulink/Sources/Repeating Sequence Interpolated  OutValues=Vst1  TimeValues=Tst1  LookUpMeth=Interpolation-Use End Values  tsamp=Tstsp  OutMin=[]  OutMax=[]  OutDataTypeStr=double  OutputDataTypeScalingMode=double  OutDataType=fixdt(0,8)  OutScaling=2^-10
  V : spsVoltageMeasurementLib/Voltage Measurement  PhasorSimulation=off  OutputType=Complex  PSBequivalent=0
  + : PMIOPort  Side=Left
  - : PMIOPort  Port=2  Side=Right
  wires:
  Memory/1 -> Controlled Current Source/1
  Repeating Sequence Interpolated/1 -> Divide/2
  Divide/1 -> Memory/1
  V/1 -> Divide/1
  connections:
  Controlled Current Source/RConn1 -- -/RConn1 -- V/LConn2
  +/RConn1 -- Controlled Current Source/LConn1 -- V/LConn1

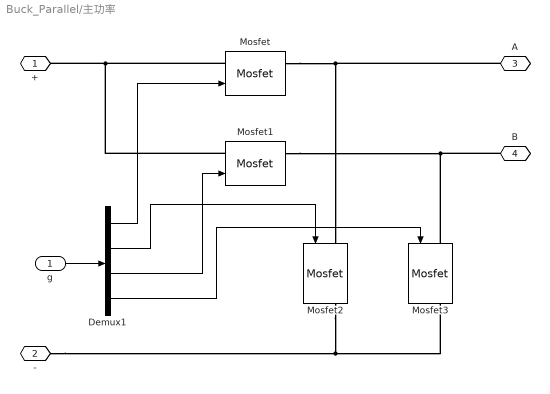
== system Buck_Parallel/主功率 ==
  g : Inport
  Demux1 : Demux
  Mosfet{,1..3} (4 alike) : spsMosfetLib/Mosfet  Ron=0.1  Lon=0  Rd=0.01  Vfd=0  IC=0  Rs=1e5  Cs=inf  Measurements=on
  + : PMIOPort  Side=Left
  - : PMIOPort  Port=2  Side=Left
  A : PMIOPort  Port=3  Side=Right
  B : PMIOPort  Port=4  Side=Right
  wires:
  g/1 -> Demux1/1
  Demux1/1 -> Mosfet/1
  Demux1/2 -> Mosfet2/1
  Demux1/3 -> Mosfet1/1
  Demux1/4 -> Mosfet3/1
  connections:
  Mosfet/RConn1 -- Mosfet2/LConn1 -- A/RConn1
  +/RConn1 -- Mosfet/LConn1 -- Mosfet1/LConn1
  Mosfet3/RConn1 -- -/RConn1 -- Mosfet2/RConn1
  B/RConn1 -- Mosfet3/LConn1 -- Mosfet1/RConn1

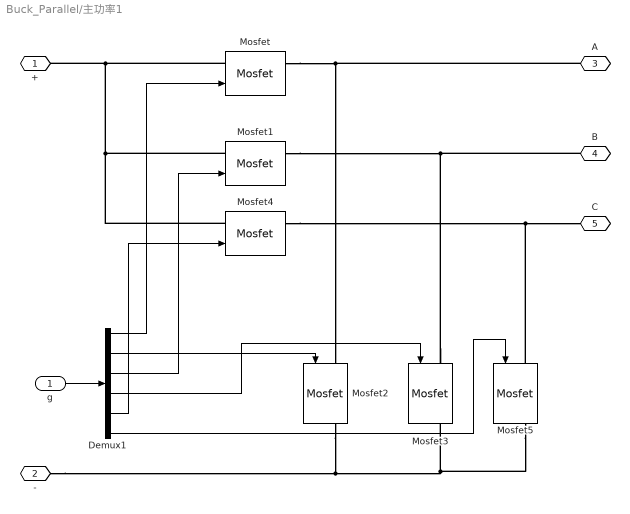
== system Buck_Parallel/主功率1 ==
  g : Inport
  Demux1 : Demux  Outputs=6
  Mosfet{,1..5} (6 alike) : spsMosfetLib/Mosfet  Ron=0.1  Lon=0  Rd=0.01  Vfd=0  IC=0  Rs=1e5  Cs=inf  Measurements=on
  + : PMIOPort  Side=Left
  - : PMIOPort  Port=2  Side=Left
  A : PMIOPort  Port=3  Side=Right
  B : PMIOPort  Port=4  Side=Right
  C : PMIOPort  Port=5  Side=Right
  wires:
  Demux1/4 -> Mosfet3/1
  Demux1/3 -> Mosfet1/1
  Demux1/2 -> Mosfet2/1
  Demux1/1 -> Mosfet/1
  g/1 -> Demux1/1
  Demux1/5 -> Mosfet4/1
  Demux1/6 -> Mosfet5/1
  connections:
  Mosfet1/RConn1 -- Mosfet3/LConn1 -- B/RConn1
  Mosfet2/RConn1 -- -/RConn1 -- Mosfet5/RConn1 -- Mosfet3/RConn1
  Mosfet1/LConn1 -- Mosfet/LConn1 -- +/RConn1 -- Mosfet4/LConn1
  A/RConn1 -- Mosfet2/LConn1 -- Mosfet/RConn1
  Mosfet4/RConn1 -- Mosfet5/LConn1 -- C/RConn1

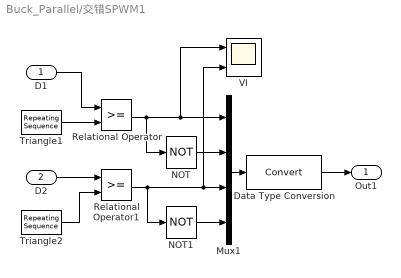
== system Buck_Parallel/交错SPWM1 ==
  D1 : Inport
  D2 : Inport  Port=2
  Data Type Conversion : DataTypeConversion  SaturateOnIntegerOverflow=off  RndMeth=Floor
  Mux1 : Mux
  NOT : Logic  Operator=NOT  IconShape=distinctive  AllPortsSameDT=off  OutDataTypeStr=boolean
  NOT1 : Logic  Operator=NOT  IconShape=distinctive  AllPortsSameDT=off  OutDataTypeStr=boolean
  Relational Operator : RelationalOperator  OutDataTypeStr=boolean  InputSameDT=off
  Relational Operator1 : RelationalOperator  OutDataTypeStr=boolean  InputSameDT=off
  Triangle1 : simulink/Sources/Repeating Sequence  rep_seq_t=[0 1/40000/2 1/40000]  rep_seq_y=[0 1 0]
  Triangle2 : simulink/Sources/Repeating Sequence  rep_seq_t=[0 1/40000/2 1/40000]  rep_seq_y=[1 0 1]
  VI : Scope  NumInputPorts=2
  Out1 : Outport
  wires:
  D1/1 -> Relational Operator/1
  NOT/1 -> Mux1/2
  D2/1 -> Relational Operator1/1
  NOT1/1 -> Mux1/4
  Triangle1/1 -> Relational Operator/2
  Mux1/1 -> Data Type Conversion/1
  Data Type Conversion/1 -> Out1/1
  Relational Operator1/1 -> Mux1/3, VI/2, NOT1/1
  Triangle2/1 -> Relational Operator1/2
  Relational Operator/1 -> Mux1/1, VI/1, NOT/1

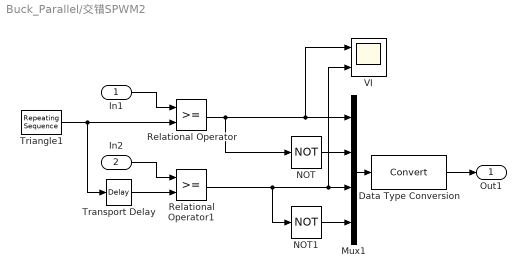
== system Buck_Parallel/交错SPWM2 ==
  In1 : Inport
  In2 : Inport  Port=2
  Data Type Conversion : DataTypeConversion  SaturateOnIntegerOverflow=off  RndMeth=Floor
  Mux1 : Mux
  NOT : Logic  Operator=NOT  IconShape=distinctive  AllPortsSameDT=off  OutDataTypeStr=boolean
  NOT1 : Logic  Operator=NOT  IconShape=distinctive  AllPortsSameDT=off  OutDataTypeStr=boolean
  Relational Operator : RelationalOperator  OutDataTypeStr=boolean  InputSameDT=off
  Relational Operator1 : RelationalOperator  OutDataTypeStr=boolean  InputSameDT=off
  Transport Delay : TransportDelay  DelayTime=1/40000/2
  Triangle1 : simulink/Sources/Repeating Sequence  rep_seq_t=[0 1/40000/2 1/40000]  rep_seq_y=[0 1 0]
  VI : Scope  NumInputPorts=2
  Out1 : Outport
  wires:
  In1/1 -> Relational Operator/1
  NOT/1 -> Mux1/2
  In2/1 -> Relational Operator1/1
  NOT1/1 -> Mux1/4
  Triangle1/1 -> Transport Delay/1, Relational Operator/2
  Mux1/1 -> Data Type Conversion/1
  Data Type Conversion/1 -> Out1/1
  Relational Operator1/1 -> Mux1/3, VI/2, NOT1/1
  Relational Operator/1 -> Mux1/1, VI/1, NOT/1
  Transport Delay/1 -> Relational Operator1/2

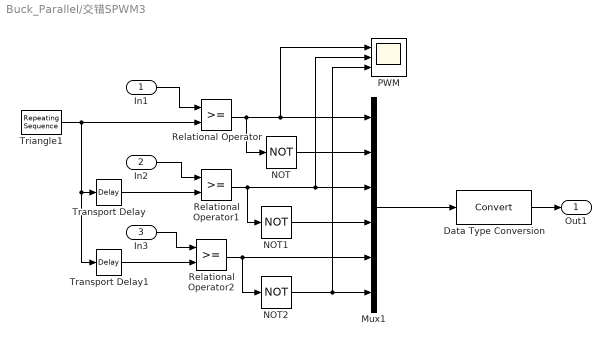
== system Buck_Parallel/交错SPWM3 ==
  In1 : Inport
  In2 : Inport  Port=2
  In3 : Inport  Port=3
  Data Type Conversion : DataTypeConversion  SaturateOnIntegerOverflow=off  RndMeth=Floor
  Mux1 : Mux  Inputs=6
  NOT : Logic  Operator=NOT  IconShape=distinctive  AllPortsSameDT=off  OutDataTypeStr=boolean
  NOT1 : Logic  Operator=NOT  IconShape=distinctive  AllPortsSameDT=off  OutDataTypeStr=boolean
  NOT2 : Logic  Operator=NOT  IconShape=distinctive  AllPortsSameDT=off  OutDataTypeStr=boolean
  PWM : Scope  NumInputPorts=3
  Relational Operator : RelationalOperator  OutDataTypeStr=boolean  InputSameDT=off
  Relational Operator1 : RelationalOperator  OutDataTypeStr=boolean  InputSameDT=off
  Relational Operator2 : RelationalOperator  OutDataTypeStr=boolean  InputSameDT=off
  Transport Delay : TransportDelay  DelayTime=1/40000/3
  Transport Delay1 : TransportDelay  DelayTime=2/40000/3
  Triangle1 : simulink/Sources/Repeating Sequence  rep_seq_t=[0 1/40000/2 1/40000]  rep_seq_y=[0 1 0]
  Out1 : Outport
  wires:
  Relational Operator/1 -> NOT/1, PWM/1, Mux1/1
  Transport Delay/1 -> Relational Operator1/2
  Relational Operator1/1 -> Mux1/3, PWM/2, NOT1/1
  Data Type Conversion/1 -> Out1/1
  Mux1/1 -> Data Type Conversion/1
  Triangle1/1 -> Transport Delay1/1, Transport Delay/1, Relational Operator/2
  NOT1/1 -> Mux1/4
  In2/1 -> Relational Operator1/1
  NOT/1 -> Mux1/2
  In1/1 -> Relational Operator/1
  Relational Operator2/1 -> NOT2/1, Mux1/5
  Transport Delay1/1 -> Relational Operator2/2
  NOT2/1 -> PWM/3, Mux1/6
  In3/1 -> Relational Operator2/1

== matlab function Buck_Parallel/MATLAB Function1 ==
  data: Vin input; D output; Vout input; iLK input; Iref input
function D = BUCK_MPC_I(Vin, Vout, iLK, Iref)
% 输出: D (占空比，范围 0-1)

% 1. 参数定义 (必须与电路一致)
Ts = 1/40000;  % 控制周期/PWM周期
L  = 1e-4;      % 电感 1mH
RL = 0.4;       % 电感内阻

% 2. 防止除零错误 (如果Vin还没上电，避免报错)
if Vin < 0.1
    D = 0;
    return;
end

% 3. 无差拍控制核心公式 (Deadbeat Control)
% 反推：为了让 iLK 在 Ts 时间后变为 Iref，需要多大的平均电压？
% 公式拆解：
% delta_I = Iref - iLK;           % 还需要补多少电流
% V_L_req = L * delta_I / Ts;     % 电感两端需要的电压
% V_in_req = V_L_req + Vout + iLK*RL; % 逆推需要的输入侧电压
% D_calc = V_in_req / Vin;        % 归一化为占空比

% 写成一行代码如下：
D_calc = (L * (Iref - iLK) / Ts + Vout + iLK * RL) / Vin;

% 4. 占空比限幅 (Saturation)
% 计算值可能 >1 或 <0，必须限制在物理可行范围内
if D_calc > 0.95        %通常留一点余量，或者直接写 1
    D = 0.95;
elseif D_calc < 0
    D = 0;
else
    D = D_calc;
end

== matlab function Buck_Parallel/MATLAB Function ==
  data: Vin input; D output; Vout input; iLK input; Iref input
function D = BUCK_MPC_I(Vin, Vout, iLK, Iref)
% 输出: D (占空比，范围 0-1)

% 1. 参数定义 (必须与电路一致)
Ts = 1/40000;  % 控制周期/PWM周期
L  = 1e-4;      % 电感 1mH
RL = 0.2;       % 电感内阻

% 2. 防止除零错误 (如果Vin还没上电，避免报错)
if Vin < 0.1
    D = 0;
    return;
end

% 3. 无差拍控制核心公式 (Deadbeat Control)
% 反推：为了让 iLK 在 Ts 时间后变为 Iref，需要多大的平均电压？
% 公式拆解：
% delta_I = Iref - iLK;           % 还需要补多少电流
% V_L_req = L * delta_I / Ts;     % 电感两端需要的电压
% V_in_req = V_L_req + Vout + iLK*RL; % 逆推需要的输入侧电压
% D_calc = V_in_req / Vin;        % 归一化为占空比

% 写成一行代码如下：
D_calc = (L * (Iref - iLK) / Ts + Vout + iLK * RL) / Vin;

% 4. 占空比限幅 (Saturation)
% 计算值可能 >1 或 <0，必须限制在物理可行范围内
if D_calc > 0.95        %通常留一点余量，或者直接写 1
    D = 0.95;
elseif D_calc < 0
    D = 0;
else
    D = D_calc;
end
